simulink model "TD2simu"  (R2024b)
settings: Solver=ode23t  StartTime=0.0  StopTime=5  RelTol=1e-3
values from neighbouring files (symbols this model uses):
  J = 0.5    [ABS.m]    (also in EBD.m; TD1_2_3.m = 0.2)
  K = 0.9    [TD1_2_3.m]
  Kd = 0    [ABS.m]    (also in EBD.m)
  Ki = 20    [ABS.m]    (also in EBD.m = 0)
  Kp = 50    [ABS.m]    (also in EBD.m = 1; TD1_2_3.m = 20)
  L = 3    [EBD.m]    (also in TD1_2_3.m = 0.01216)
  R = 0.895    [TD1_2_3.m]
undefined symbols (not defined in the file or in its folder): b, Cr
libraries: simulink x1
settings Model: Creator=E306-PC2  LastModifiedBy=julien.dbc

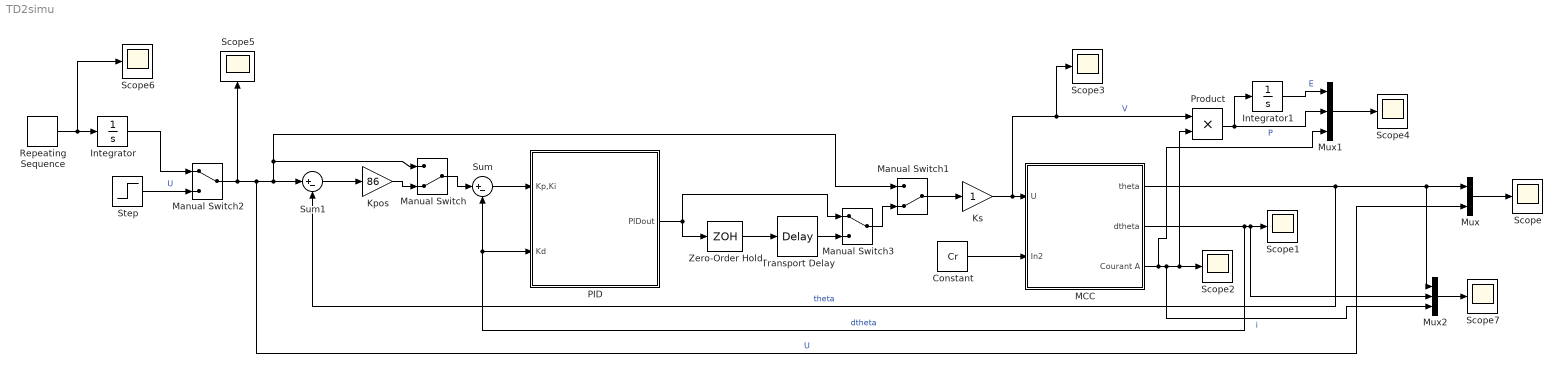
== system TD2simu ==
  Constant : Constant  Value=Cr
  Integrator : Integrator
  Integrator1 : Integrator
  Kpos : Gain  Gain=86
  Ks : Gain
  MCC : Subsystem
  Manual Switch : ManualSwitch  CurrentSetting=0
  Manual Switch1 : ManualSwitch  CurrentSetting=0
  Manual Switch2 : ManualSwitch
  Manual Switch3 : ManualSwitch
  Mux : Mux  Inputs=2
  Mux1 : Mux  Inputs=3
  Mux2 : Mux  Inputs=3
  PID : Subsystem
  Product : Product
  Repeating Sequence : simulink/Sources/Repeating Sequence  rep_seq_t=[0 0.05 0.25 0.3 5]  rep_seq_y=[0 40 40 0 0]
  Scope{,1..7} (8 alike) : Scope
  Step : Step  Time=0  SampleTime=0
  Sum : Sum  Inputs=|+-
  Sum1 : Sum  Inputs=|+-
  Transport Delay : TransportDelay  DelayTime=0.002
  Zero-Order Hold : ZeroOrderHold  SampleTime=1/250
  wires:
  Constant/1 -> MCC/2(In2)
  MCC/1(theta) -> Mux/1, Mux2/1, Sum1/2  "theta"
  Manual Switch1/1 -> Ks/1
  Sum1/1 -> Kpos/1
  Manual Switch/1 -> Sum/1
  MCC/3(Courant A) -> Mux1/3, Mux2/3, Scope2/1, Product/2  "i"
  Kpos/1 -> Manual Switch/2
  Ks/1 -> Scope3/1, Product/1, MCC/1(U)  "V"
  Manual Switch2/1 -> Mux/2, Sum1/1, Manual Switch/1, Manual Switch1/1, Scope5/1  "U"
  Step/1 -> Manual Switch2/2  "U"
  Integrator/1 -> Manual Switch2/1
  Repeating Sequence/1 -> Scope6/1, Integrator/1
  Product/1 -> Mux1/2, Integrator1/1  "P"
  Mux/1 -> Scope/1
  Integrator1/1 -> Mux1/1  "E"
  Mux1/1 -> Scope4/1
  MCC/2(dtheta) -> Mux2/2, Scope1/1, Sum/2, PID/2(Kd)  "dtheta"
  Sum/1 -> PID/1(Kp,Ki)
  Zero-Order Hold/1 -> Transport Delay/1
  PID/1(PIDout) -> Zero-Order Hold/1, Manual Switch3/1
  Transport Delay/1 -> Manual Switch3/2
  Manual Switch3/1 -> Manual Switch1/2
  Mux2/1 -> Scope7/1

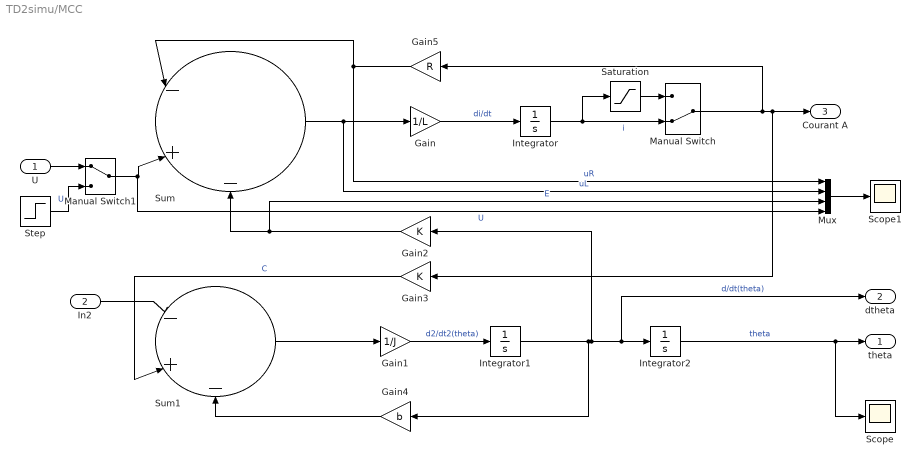
== system TD2simu/MCC ==
  U : Inport
  In2 : Inport  Port=2
  Gain : Gain  Gain=1/L
  Gain1 : Gain  Gain=1/J
  Gain2 : Gain  Gain=K
  Gain3 : Gain  Gain=K
  Gain4 : Gain  Gain=b
  Gain5 : Gain  Gain=R
  Integrator : Integrator
  Integrator1 : Integrator
  Integrator2 : Integrator
  Manual Switch : ManualSwitch  CurrentSetting=0
  Manual Switch1 : ManualSwitch
  Mux : Mux
  Saturation : Saturate  UpperLimit=20  LowerLimit=-20
  Scope : Scope
  Scope1 : Scope
  Step : Step  Time=0  After=12  SampleTime=0
  Sum : Sum  Inputs=|-+-
  Sum1 : Sum  Inputs=|-+-
  theta : Outport
  dtheta : Outport  Port=2
  Courant A : Outport  Port=3
  wires:
  Mux/1 -> Scope1/1
  Sum/1 -> Mux/2, Gain/1  "uL"
  Gain5/1 -> Sum/1, Mux/1  "uR"
  Sum1/1 -> Gain1/1
  Gain1/1 -> Integrator1/1  "d2/dt2(theta)"
  Gain2/1 -> Mux/3, Sum/3  "E"
  Gain4/1 -> Sum1/3
  Gain3/1 -> Sum1/2  "C"
  Integrator1/1 -> Gain4/1, Gain2/1, dtheta/1, Integrator2/1  "d/dt(theta)"
  Integrator/1 -> Saturation/1, Manual Switch/2  "i"
  In2/1 -> Sum1/1
  Gain/1 -> Integrator/1  "di/dt"
  Integrator2/1 -> Scope/1, theta/1  "theta"
  Manual Switch/1 -> Gain3/1, Courant A/1, Gain5/1
  Saturation/1 -> Manual Switch/1
  U/1 -> Manual Switch1/1
  Manual Switch1/1 -> Mux/4, Sum/2  "U"
  Step/1 -> Manual Switch1/2  "U"

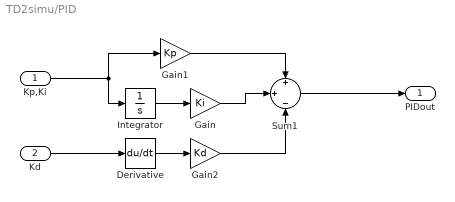
== system TD2simu/PID ==
  Kp,Ki : Inport
  Kd : Inport  Port=2
  Derivative : Derivative  CoefficientInTFapproximation=0.001
  Gain : Gain  Gain=Ki
  Gain1 : Gain  Gain=Kp
  Gain2 : Gain  Gain=Kd
  Integrator : Integrator
  Sum1 : Sum  Inputs=+|+|-
  PIDout : Outport
  wires:
  Gain2/1 -> Sum1/3
  Derivative/1 -> Gain2/1
  Integrator/1 -> Gain/1
  Gain1/1 -> Sum1/1
  Gain/1 -> Sum1/2
  Sum1/1 -> PIDout/1
  Kp,Ki/1 -> Integrator/1, Gain1/1
  Kd/1 -> Derivative/1
